simulink library "driver_maneuver_library"  (R2025a)
settings: Solver=VariableStepAuto  StartTime=0.0  StopTime=10.0  RelTol=1e-3
libraries: simulink_extras x1, slpidlib x1
Description:
  | Copyright 2021-2025 The MathWorks, Inc.
settings Model: Creator=smiller  LastModifiedBy=smiller
settings SolverCC: AlgebraicLoopSolver=TrustRegion
settings OptimizationCC: ReuseModelBlockBuffer=off
settings DebuggingCC: UnconnectedInputMsg=warning  UnconnectedOutputMsg=warning  UnconnectedLineMsg=warning
settings ModelReferenceCC: EnableRefExpFcnMdlSchedulingChecks=on
settings RTWCC: GPUComputeCapability=3.5  DLArmComputeVersion=19.05

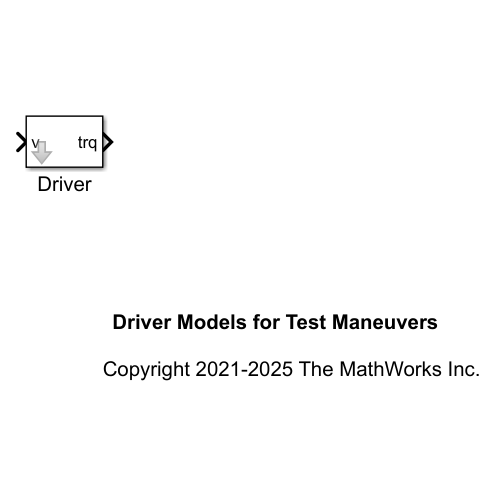
[thumbnail: Simulink's stored preview of the top-level diagram]
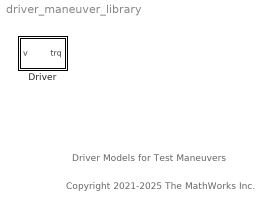
== system driver_maneuver_library ==
  note: Driver Models for Test Maneuvers
  note: Copyright 2021-2025 The MathWorks Inc.
  Driver : Subsystem  mask(Human Driver Model){max_torque=200, spd_cruise_1=100, spd_other_car=80, initial_lead_dist=100, follow_dist=40, pass_start_time=180, spd_passing=160, lead_dist=20, spd_cruise_2=100}
      mask prompts: max_torque "Full throttle torque (N*m):"; spd_cruise_1 "Initial cruise speed (km/hr)"; spd_other_car "Slower car cruise speed (km/hr)"; initial_lead_dist "Initial follow distance (m)"; follow_dist "Minimum follow distance (m)"; pass_start_time "Lane change initiation time (s)"; spd_passing "Passing lane speed (km/hr)"; lead_dist "Minimum lead distance (m)"; spd_cruise_2 "Final cruise speed (km/hr)"
      mask help:
      | This block represents a driver executing a passing maneuver.
      |
      | The single input, v, is the forward velocity of the subject vehicle. The output is the amount of torque the driver is requesting from the motor to complete the maneuver.
      mask DialogControl primary_tab Prompt: Driver Input
      mask DialogControl secondary_tab Prompt: Behavior

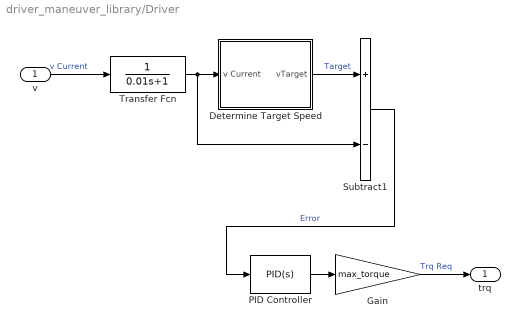
== system driver_maneuver_library/Driver ==
  v : Inport
  Determine Target Speed : Subsystem
  Gain : Gain  Gain=max_torque
  PID Controller : slpidlib/PID Controller  Controller=PID  Form=Parallel  TimeDomain=Continuous-time  UseExternalTs=off  SampleTime=-1  IntegratorMethod=Forward Euler  FilterMethod=Forward Euler  ControllerParametersSource=internal  P=1e-1  I=1e-1  UseKiTs=off  D=1e-3  UseExternalDerivativeSource=off  N=100  UseFilter=on  TunerSelectOption=Transfer Function Based (PID Tuner App)  InitialConditionSource=internal  InitialConditionForIntegrator=0  InitialConditionForFilter=0  DifferentiatorICPrevScaledInput=0  ExternalReset=none  TrackingMode=off  Kt=1  LimitOutput=on  SatLimitsSource=internal  UpperSaturationLimit=1  LowerSaturationLimit=-1  LinearizeAsGain=off  AntiWindupMode=back-calculation  Kb=1  LimitIntegrator=off  UpperIntegratorSaturationLimit=inf  LowerIntegratorSaturationLimit=-inf  POutMin=[]  POutMax=[]  IOutMin=[]  IOutMax=[]  DOutMin=[]  DOutMax=[]  NOutMin=[]  NOutMax=[]  SumOutMin=[]  SumOutMax=[]  SaturationOutMin=[]  SaturationOutMax=[]  PParamMin=[]  PParamMax=[]  IParamMin=[]  IParamMax=[]  DParamMin=[]  DParamMax=[]  NParamMin=[]  NParamMax=[]  KbParamMin=[]  KbParamMax=[]  KtParamMin=[]  KtParamMax=[]  KbOutMin=[]  KbOutMax=[]  KtOutMin=[]  KtOutMax=[]  IntegratorOutMin=[]  IntegratorOutMax=[]  FilterOutMin=[]  FilterOutMax=[]  SumI1OutMin=[]  SumI1OutMax=[]  SumI2OutMin=[]  SumI2OutMax=[]  SumI3OutMin=[]  SumI3OutMax=[]  SumI4OutMin=[]  SumI4OutMax=[]  SumDOutMin=[]  SumDOutMax=[]  DifferentiatorOutMin=[]  DifferentiatorOutMax=[]  FilterDiffOutCoefMin=[]  FilterDiffOutCoefMax=[]  ReciprocalOutMin=[]  ReciprocalOutMax=[]  SumDenOutMin=[]  SumDenOutMax=[]  SumNumOutMin=[]  SumNumOutMax=[]  DivideOutMin=[]  DivideOutMax=[]  UdiffTsProdOutMin=[]  UdiffTsProdOutMax=[]  NTsProdOutMin=[]  NTsProdOutMax=[]  UintegralTsProdOutMin=[]  UintegralTsProdOutMax=[]  UngainTsProdOutMin=[]  UngainTsProdOutMax=[]  ClampingZeroOutDataTypeStr=Inherit: Inherit via back propagation  ClampingZeroOutMin=[]  ClampingZeroOutMax=[]  FilterDenConstantOutDataTypeStr=Inherit: Inherit via back propagation  FilterDenConstantOutMin=[]  FilterDenConstantOutMax=[]  PCopyOutDataTypeStr=Inherit: Inherit via back propagation  PCopyOutMin=[]  PCopyOutMax=[]  NCopyOutDataTypeStr=Inherit: Inherit via back propagation  NCopyOutMin=[]  NCopyOutMax=[]  IntegratorContinuousStateAttributes=''  IntegratorStateMustResolveToSignalObject=off  IntegratorRTWStateStorageClass=Auto  FilterContinuousStateAttributes=''  FilterStateMustResolveToSignalObject=off  FilterRTWStateStorageClass=Auto  ParallelPVariant=InternalParameters  IdealPVariant=Disabled  IVariant=InternalParameters  DVariant=InternalParameters  IntegratorVariant=Continuous  SatVariant=Enabled  AWVariant=BackCalculation  PCopyVariant=Disabled  TRVariant=Disabled  FdbkBlocksVariant=Forward  IdealPFdbkVariant=Disabled  SatFdbkVariant=Disabled  DerivativeFilterVariant=ContFilter  NVariant=InternalParameters  NCopyVariant=Disabled  FilterICVariant=InternalICsFilter  IntegratorICVariant=InternalICs  ExternalResetVariant=Disabled  TRSumVariant=Passthrough  SumFdbkVariant=Disabled  SumVariant=Sum_PID  TsampFilterVariant=InternalTs  TsampNgainVariant=Passthrough  TsampIntegralVariant=Disabled_SignalSpec  ExternalSaturationOutDataTypeStr=Inherit: Same as second input  DerivativeSourceVariant=ErrorSignal  PreIntVariant=InternalPreInt
  Subtract1 : Sum  Inputs=+-
  Transfer Fcn : TransferFcn  Denominator=[0.01 1]
  trq : Outport
  wires:
  v/1 -> Transfer Fcn/1  "v Current"
  Gain/1 -> trq/1  "Trq Req"
  Subtract1/1 -> PID Controller/1  "Error"
  PID Controller/1 -> Gain/1
  Determine Target Speed/1(vTarget) -> Subtract1/1  "Target"
  Transfer Fcn/1 -> Determine Target Speed/1(v Current), Subtract1/2

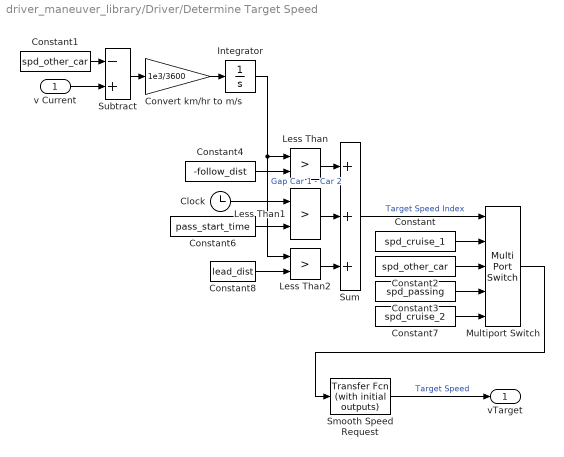
== system driver_maneuver_library/Driver/Determine Target Speed ==
  v Current : Inport
  Clock : Clock
  Constant : Constant  Value=spd_cruise_1
  Constant1 : Constant  Value=spd_other_car
  Constant2 : Constant  Value=spd_other_car
  Constant3 : Constant  Value=spd_passing
  Constant4 : Constant  Value=-follow_dist
  Constant6 : Constant  Value=pass_start_time
  Constant7 : Constant  Value=spd_cruise_2
  Constant8 : Constant  Value=lead_dist
  Convert km/hr to m/s : Gain  Gain=1e3/3600
  Integrator : Integrator  InitialCondition=-initial_lead_dist
  Less Than : RelationalOperator  Operator=>  OutDataTypeStr=boolean  RndMeth=Simplest  InputSameDT=off
  Less Than1 : RelationalOperator  Operator=>  OutDataTypeStr=boolean  RndMeth=Simplest  InputSameDT=off
  Less Than2 : RelationalOperator  Operator=>  OutDataTypeStr=boolean  RndMeth=Simplest  InputSameDT=off
  Multiport Switch : MultiPortSwitch  DataPortOrder=Zero-based contiguous  Inputs=4  zeroidx=on  SaturateOnIntegerOverflow=off  InputSameDT=off
  Smooth Speed Request : simulink_extras/Additional Linear/Transfer Fcn (with initial outputs)  N=[1]  D="[2  1]"  Y0=spd_cruise_1  U0=spd_cruise_1
  Subtract : Sum  Inputs=-+
  Sum : Sum  Inputs=+++
  vTarget : Outport
  wires:
  Clock/1 -> Less Than1/1
  Constant/1 -> Multiport Switch/2
  Integrator/1 -> Less Than2/1, Less Than/1  "Gap Car 1 - Car 2"
  Multiport Switch/1 -> Smooth Speed Request/1
  Constant7/1 -> Multiport Switch/5
  Convert km/hr to m/s/1 -> Integrator/1
  Subtract/1 -> Convert km/hr to m/s/1
  Sum/1 -> Multiport Switch/1  "Target Speed Index"
  Constant3/1 -> Multiport Switch/4
  Less Than/1 -> Sum/1
  Less Than2/1 -> Sum/3
  Less Than1/1 -> Sum/2
  Constant6/1 -> Less Than1/2
  Constant1/1 -> Subtract/1
  Constant4/1 -> Less Than/2
  Constant2/1 -> Multiport Switch/3
  Constant8/1 -> Less Than2/2
  Smooth Speed Request/1 -> vTarget/1  "Target Speed"
  v Current/1 -> Subtract/2
